simulink model "FZ"  (R2024b)
settings: Solver=ode3  StartTime=0.0  StopTime=100  FixedStep=0.01  RelTol=1e-3
settings Model: Creator=liuhelai  LastModifiedBy=liuhelai

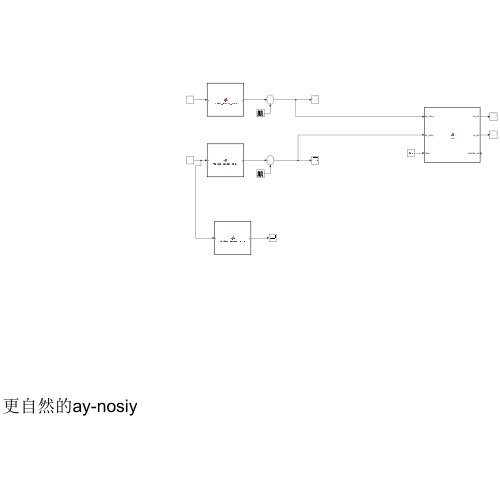
[thumbnail: Simulink's stored preview of the top-level diagram]
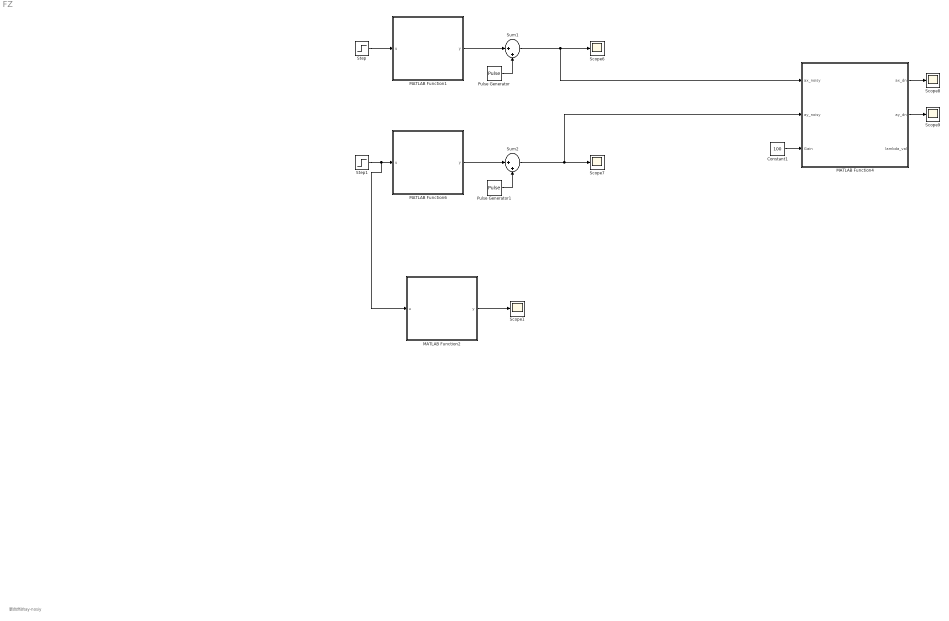
== system FZ ==
  note: 更自然的ay-nosiy
  Constant1 : Constant  Value=100
  MATLAB Function1 : MATLAB Function  TreatAsAtomicUnit=on  SystemSampleTime=0.01
  MATLAB Function2 : MATLAB Function  TreatAsAtomicUnit=on  SystemSampleTime=0.01
  MATLAB Function4 : MATLAB Function  TreatAsAtomicUnit=on
  MATLAB Function6 : MATLAB Function  TreatAsAtomicUnit=on  SystemSampleTime=0.01
  Pulse Generator : DiscretePulseGenerator  PulseType=Time based  Amplitude=0.26  Period=1000  PulseWidth=0.01  PhaseDelay=10.76
  Pulse Generator1 : DiscretePulseGenerator  PulseType=Time based  Amplitude=-0.36  Period=1000  PulseWidth=0.01  PhaseDelay=10.76
  Scope{1,6..9} (5 alike) : Scope
  Step : Step  SampleTime=0
  Step1 : Step  SampleTime=0
  Sum1 : Sum  Inputs=|++
  Sum2 : Sum  Inputs=|++
  wires:
  Step/1 -> MATLAB Function1/1(u)
  MATLAB Function1/1(y) -> Sum1/1
  Sum1/1 -> MATLAB Function4/1(ax_noisy), Scope6/1
  Pulse Generator/1 -> Sum1/2
  Pulse Generator1/1 -> Sum2/2
  Sum2/1 -> MATLAB Function4/2(ay_noisy), Scope7/1
  MATLAB Function6/1(y) -> Sum2/1
  Step1/1 -> MATLAB Function2/1(u), MATLAB Function6/1(u)
  Constant1/1 -> MATLAB Function4/3(Gain)
  MATLAB Function4/1(ax_dn) -> Scope8/1
  MATLAB Function4/2(ay_dn) -> Scope9/1
  MATLAB Function2/1(y) -> Scope1/1

== matlab function FZ/MATLAB Function1 ==
  data: u input; y output
function y = realistic_sensor_noise(u)


% ---目标参数 ---
    sigma_desired = 0.053721; % 标准差
    mu = 0.003058;   
alpha = 0.85;            % 平滑系数
drift_strength = 0.0002; % 漂移

% --- 2. 状态保存 ---
persistent last_noise drift_val is_initialized
if isempty(is_initialized)
    last_noise = 0;
    drift_val = 0;
    is_initialized = 1;
end

% --- 3. 核心计算 ---

% 计算能量补偿增益
K = sqrt((1 + alpha) / (1 - alpha));

% 生成原始白噪声并滤波
raw_white = sigma_desired * randn();
filtered_noise = (1 - alpha) * raw_white + alpha * last_noise;
last_noise = filtered_noise;

% 加上补偿增益
natural_noise = filtered_noise * K;

% 随机游走漂移
drift_val = drift_val + drift_strength * randn();

% 合成输出
y = u + mu + natural_noise + drift_val;

== matlab function FZ/MATLAB Function2 ==
  data: u input; y output
function y = realistic_sensor_noise(u)


% --- 1. 目标参数 ---
    sigma_desired = 0.00002; % 标准差
    mu = 0.00004;    
alpha = 0.95;            % 平滑系数
drift_strength = 0.0002; % 漂移

% --- 2. 状态保存 ---
persistent last_noise drift_val is_initialized
if isempty(is_initialized)
    last_noise = 0;
    drift_val = 0;
    is_initialized = 1;
end

% --- 3. 核心计算 ---

% 计算能量补偿增益
K = sqrt((1 + alpha) / (1 - alpha));

% 生成原始白噪声并滤波
raw_white = sigma_desired * randn();
filtered_noise = (1 - alpha) * raw_white + alpha * last_noise;
last_noise = filtered_noise;

% 加上补偿增益
natural_noise = filtered_noise * K;

% 随机游走漂移
drift_val = drift_val + drift_strength * randn();

% 合成输出
y = u + mu + natural_noise + drift_val;

== matlab function FZ/MATLAB Function4 ==
  data: ax_noisy input; ax_dn output; ay_noisy input; ay_dn output; lambda_val output; Gain input
function [ax_dn, ay_dn, lambda_val] = fcn(ax_noisy, ay_noisy, Gain)


persistent buffer_ax buffer_ay
window_size = 64; % 支持多层分解
if isempty(buffer_ax)
    buffer_ax = zeros(window_size, 1);
    buffer_ay = zeros(window_size, 1);
end

% 1. 更新滑动窗口
buffer_ax = [buffer_ax(2:end); ax_noisy];
buffer_ay = [buffer_ay(2:end); ay_noisy];

% --- 2. 改进的工况自适应算子 ---
curr_std = std(buffer_ax);
alpha = 1 / (1 + exp(20 * (curr_std - 0.5))); 

% --- 3. 3层离散小波分解 (Haar) ---
x = buffer_ax;
y = buffer_ay;

% 第一层
[A1x, D1x] = haar_dec(x);
[A1y, D1y] = haar_dec(y);
% 第二层
[A2x, D2x] = haar_dec(A1x);
[A2y, D2y] = haar_dec(A1y);
% 第三层
[A3x, D3x] = haar_dec(A2x);
[A3y, D3y] = haar_dec(A2y);

% --- 4. 阈值计算  ---
sigma_est = median(abs(D1x)) / 0.6745;
if sigma_est < 0.001, sigma_est = std(D1x); end 

% 核心阈值公式
lambda = Gain * sigma_est * sqrt(2 * log(window_size)) * (0.5 + 0.5*alpha);
lambda_val = lambda;

% --- 5. 执行去噪 ---
D1x_t = mod_thr(D1x, lambda);   D1y_t = mod_thr(D1y, lambda);
D2x_t = mod_thr(D2x, lambda*1.2); D2y_t = mod_thr(D2y, lambda*1.2);
D3x_t = mod_thr(D3x, lambda*1.5); D3y_t = mod_thr(D3y, lambda*1.5);

% --- 6. 多层重构 ---
R2x = haar_rec(A3x, D3x_t); R2y = haar_rec(A3y, D3y_t);
R1x = haar_rec(R2x, D2x_t); R1y = haar_rec(R2y, D2y_t);
final_x = haar_rec(R1x, D1x_t); final_y = haar_rec(R1y, D1y_t);

% 输出重构序列的最后一个点
ax_dn = final_x(end);
ay_dn = final_y(end);

end

% --- Haar分解 ---
function [A, D] = haar_dec(sig)
    N = length(sig);
    A = zeros(N/2, 1);
    D = zeros(N/2, 1);
    for i = 1:N/2
        A(i) = (sig(2*i-1) + sig(2*i)) / 1.4142;
        D(i) = (sig(2*i-1) - sig(2*i)) / 1.4142;
    end
end

% --- Haar重构 ---
function sig = haar_rec(A, D)
    N2 = length(A);
    sig = zeros(N2*2, 1);
    for i = 1:N2
        sig(2*i-1) = (A(i) + D(i)) / 1.4142;
        sig(2*i)   = (A(i) - D(i)) / 1.4142;
    end
end

% --- 改进阈值函数 ---
function d_thr = mod_thr(d, lam)
    d_thr = zeros(size(d));
    k = 2.0; 
    for i = 1:length(d)
        if abs(d(i)) > lam
            % 使用更具收缩力的阈值函数
            d_thr(i) = sign(d(i)) * (abs(d(i)) - 0.8 * lam / exp(k * (abs(d(i)) - lam)));
        else
            d_thr(i) = 0;
        end
    end
end

== matlab function FZ/MATLAB Function6 ==
  data: u input; y output
function y = realistic_sensor_noise(u)


% --- 1. 目标参数 ---
    sigma_desired = 0.05432; % 标准差
    mu = 0.00514;    
alpha = 0.75;            % 平滑系数 
drift_strength = 0.001; % 漂移

% --- 2. 状态保存 ---
persistent last_noise drift_val is_initialized
if isempty(is_initialized)
    last_noise = 0;
    drift_val = 0;
    is_initialized = 1;
end

% --- 3. 核心计算 ---

% 计算能量补偿增益
K = sqrt((1 + alpha) / (1 - alpha));

% 生成原始白噪声并滤波
raw_white = sigma_desired * randn();
filtered_noise = (1 - alpha) * raw_white + alpha * last_noise;
last_noise = filtered_noise;

%加上补偿增益
natural_noise = filtered_noise * K;

% 随机游走漂移
drift_val = drift_val + drift_strength * randn();

%合成输出
y = u + mu + natural_noise + drift_val;
